simulink model "Ackermann_Env"  (R2025a)
settings: Solver=FixedStepAuto  StartTime=0.0  RelTol=1e-3
values from neighbouring files (symbols this model uses):
  dist0 = sqrt((pathXY_padded(end,1)-x0)^2 + (pathXY_padded(end,2)-y0)^2)    [testing_sebelum_v3.m]    (also in testing_v2.m)
  pathXY_padded = zeros(MAX_PATH_SIZE, 2)    [pad_path.m]    (also in pad_path_old.m = [pathXY; pad]; testing_sebelum_v3.m = pad_path(pathXY_raw, MAX_PATH_SIZE); testing_v2.m = pad_path(pathXY_raw, MAX_PATH_SIZE))
  slip_factor = 1.0    (= 1)    [testing_sebelum_v3.m]
undefined symbols (not defined in the file or in its folder): idx0
libraries: ros2lib x2, rllib x1
settings Model: Creator=raka-argha  LastModifiedBy=raka-argha
settings OptimizationCC: DefaultParameterBehavior=Inlined  EnhancedBackFolding=on  PassReuseOutputArgsAs=Individual arguments  ZeroExternalMemoryAtStartup=off  ZeroInternalMemoryAtStartup=off  MaxStackSize=64  OptimizeBlockOrder=speed  DifferentSizesBufferReuse=on  OptimizationCustomize=off  EfficientTunableParamExpr=on
settings DebuggingCC: ParameterTunabilityLossMsg=error
settings HardwareCC: ProdBitPerLong=64.0  ProdHWDeviceType=Intel->x86-64 (Linux 64)
settings SFSimCC: MATLABDynamicMemAlloc=off
settings RTWCC: SystemTargetFile=ert.tlc  HardwareBoard=Robot Operating System 2 (ROS 2)  TLCOptions="-aInlineSetEventsForThisBaseRateFcn=TLC_FALSE -aSuppressMultiTaskScheduler=TLC_FALSE  -aRateBasedStepFcn=0"  TemplateMakefile=ert_default_tmf  Toolchain=Colcon Tools  TargetLang=C++  Description=Embedded Coder
settings CodeAppCC: ForceParamTrailComments=on  IgnoreCustomStorageClasses=off  OperatorAnnotations=on  SimulinkDataObjDesc=on  SFDataObjDesc=on  InsertBlockDesc=on
settings ERTTargetCC: ExtModeTransport=2.0  RootIOFormat=Structure reference  CodeInterfacePackaging=C++ class

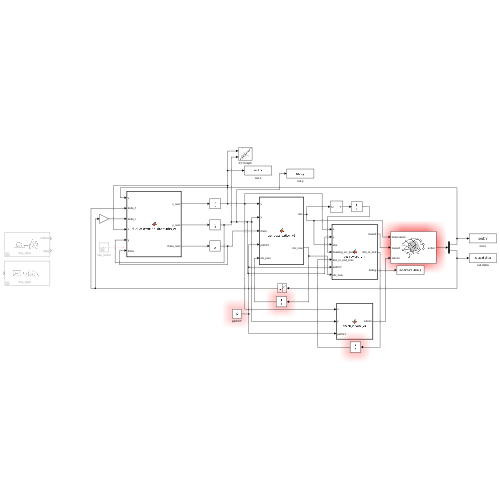
[thumbnail: Simulink's stored preview of the top-level diagram]
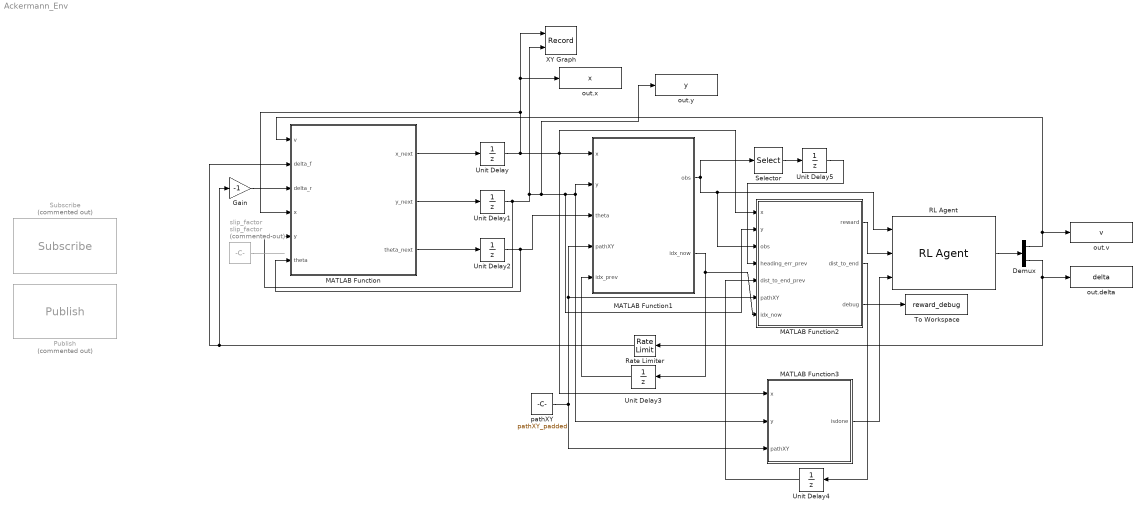
== system Ackermann_Env ==
  Demux : Demux  Outputs=2
  Gain : Gain  Gain=-1
  MATLAB Function : MATLAB Function  TreatAsAtomicUnit=on
  MATLAB Function1 : MATLAB Function  TreatAsAtomicUnit=on
  MATLAB Function2 : MATLAB Function  TreatAsAtomicUnit=on
  MATLAB Function3 : MATLAB Function  TreatAsAtomicUnit=on
  Publish : ros2lib/Publish  Commented=on  topicSource=Select from ROS network  topic=/my_topic  messageType=geometry_msgs/Point  QOSHistory=Keep last  QOSDepth=10  QOSReliability=Reliable  QOSDurability=Volatile  QOSDeadline=Inf  QOSLifespan=Inf  QOSLiveliness=Automatic  QOSLeaseDuration=Inf  QOSAvoidROSNamespaceConventions=off
  RL Agent : rllib/RL Agent  Agent=agentObj  ExternalActionAsInput=off  ProvideLastAction=off  ProvideCumRwd=off  TreatAsDirectFeedthrough=on  UseStrictObservationDataTypes=off
  Rate Limiter : RateLimiter  RisingSlewLimit=1.0  FallingSlewLimit=-1.0  SampleTimeMode=inherited
  Selector : Selector  IndexOptions=Index vector (dialog)  Indices=2  OutputSizes=1
  Subscribe : ros2lib/Subscribe  Commented=on  topicSource=Select from ROS network  topic=/my_topic  messageType=geometry_msgs/Point  sampleTime=-1  QOSHistory=Keep last  QOSDepth=10  QOSReliability=Reliable  QOSDurability=Volatile  QOSDeadline=Inf  QOSLifespan=Inf  QOSLiveliness=Automatic  QOSLeaseDuration=Inf  QOSAvoidROSNamespaceConventions=off
  To Workspace : ToWorkspace  VariableName=reward_debug  SaveFormat=Timeseries  SampleTime=-1
  Unit Delay{,1..2,5} (4 alike) : UnitDelay  SampleTime=-1  HasFrameUpgradeWarning=on
  Unit Delay3 : UnitDelay  InitialCondition=idx0  SampleTime=-1  HasFrameUpgradeWarning=on
  Unit Delay4 : UnitDelay  InitialCondition=dist0  SampleTime=-1  HasFrameUpgradeWarning=on
  XY Graph : Record  NumPorts=2.0  FileSettingsInternal="{\"entries\":[{\"content\":{\"excelSettings\":{\"content\":{},\"type\":\"Streamout.ExcelSettings\"},\"parquetSettings\":{\"content\":{},\"type\":\"Streamout.ParquetSettings\"}},\"type\":\"Streamout.FileSettingStorage\",\"uuid\":\"\"}],\"packageUris\":[\"http:\\/\\/schema.mathworks.com\\/mf0\\/streamout_blocks\\/R2020a\"],\"version\":\"1.0\"}"  FrameSettings=[0, 0]  Layout=[1 1]  SignalsInternal="{\"entries\":[{\"content\":{\"signals\":[{\"content\":{\"blockPath\":[],\"dimensions\":[1],\"domain\":\"\",\"lineColor\":\"#fe330a\",\"lineWidth\":2,\"port\":1,\"signalID\":1,\"signalName\":\"Unit Delay\"},\"type\":\"RecordBlkView.Signal\",\"uuid\":\"\"},{\"content\":{\"blockPath\":[],\"dimensions\":[1],\"domain\":\"\",\"lineColor\":\"#22b573\",\"lineWidth\":2,\"port\":2,\"signalID\":2,\"signalName\":\"Unit Delay1\"},\"type\":\"RecordBlkView.Signal\",\"uuid\":\"\"}]},\"type\":\"RecordBlkView.InputSignals\",\"uuid\":\"\"}],\"packageUris\":[\"http:\\/\\/schema.mathworks.com\\/mf0\\/streamout_blocks\\/R2020a\"],\"version\":\"1.0\"}"  VisualizationBindings="{\"xyplotplugin\":{\"info\":[{\"series\":[],\"subplotID\":1}]}}"  CompatibilityTag=XY
  out.delta : ToWorkspace  VariableName=delta  SaveFormat=Timeseries  SampleTime=-1
  out.v : ToWorkspace  VariableName=v  SaveFormat=Timeseries  SampleTime=-1
  out.x : ToWorkspace  VariableName=x  SaveFormat=Timeseries  SampleTime=-1
  out.y : ToWorkspace  VariableName=y  SaveFormat=Timeseries  SampleTime=-1
  pathXY : Constant  Value=pathXY_padded
  slip_factor : Constant  Commented=on  Value=slip_factor
  wires:
  MATLAB Function/1(x_next) -> Unit Delay/1
  MATLAB Function/2(y_next) -> Unit Delay1/1
  MATLAB Function/3(theta_next) -> Unit Delay2/1
  Unit Delay/1 -> out.x/1, XY Graph/1, MATLAB Function/4(x), MATLAB Function3/1(x), MATLAB Function2/1(x), MATLAB Function1/1(x)
  Unit Delay1/1 -> XY Graph/2, out.y/1, MATLAB Function2/2(y), MATLAB Function3/2(y), MATLAB Function1/2(y), MATLAB Function/5(y)
  Unit Delay2/1 -> MATLAB Function1/3(theta), MATLAB Function/6(theta)
  MATLAB Function1/1(obs) -> RL Agent/1, MATLAB Function2/3(obs), Selector/1
  MATLAB Function3/1(isdone) -> RL Agent/3
  MATLAB Function2/1(reward) -> RL Agent/2
  RL Agent/1 -> Demux/1
  Demux/1 -> out.v/1, MATLAB Function/1(v)
  Demux/2 -> Rate Limiter/1, out.delta/1
  Rate Limiter/1 -> Gain/1, MATLAB Function/2(delta_f)
  pathXY/1 -> MATLAB Function1/4(pathXY), MATLAB Function2/6(pathXY), MATLAB Function3/3(pathXY)
  Unit Delay4/1 -> MATLAB Function2/5(dist_to_end_prev)
  slip_factor/1 -> ?
  Selector/1 -> Unit Delay5/1
  MATLAB Function2/2(dist_to_end) -> Unit Delay4/1
  MATLAB Function2/3(debug) -> To Workspace/1
  Unit Delay5/1 -> MATLAB Function2/4(heading_err_prev)
  MATLAB Function1/2(idx_now) -> MATLAB Function2/7(idx_now), Unit Delay3/1
  Unit Delay3/1 -> MATLAB Function1/5(idx_prev)
  Gain/1 -> MATLAB Function/3(delta_r)

== matlab function Ackermann_Env/MATLAB Function1 ==
  data: x input; obs output; y input; theta input; pathXY input; idx_prev input; idx_now output
function [obs, idx_now] = get_observation_v6(x, y, theta, pathXY, idx_prev)
%#codegen
% GET_OBSERVATION_V6
%
% PERBEDAAN UTAMA DARI V5:
%   1. Index TIDAK BOLEH merayap melewati ujung path ASLI (N), bukan ujung
%      array padding (300). Ini yang dulu bikin dist_to_end jadi 0 permanen.
%   2. Observasi dinormalisasi supaya skalanya seragam (CTE ~1, waypoint ~5m
%      dibagi 5). SAC jauh lebih stabil dengan input yang sebanding.
%
% Ukuran port TIDAK BERUBAH: 5 input, 2 output, obs tetap 23x1.
% Jadi TIDAK PERLU mengubah wiring Simulink sama sekali.

    N_LOOKAHEAD = 10;
    STRIDE      = 5;
    WINDOW_BACK = 2;
    WINDOW_FWD  = 5;
    SKALA_WP    = 5.0;    % waypoint lookahead dibagi ini

    N = panjang_path_asli(pathXY);

    idx_prev = round(idx_prev);
    if idx_prev < 1, idx_prev = 1; end
    if idx_prev > N, idx_prev = N; end

    lo = max(1, idx_prev - WINDOW_BACK);
    hi = min(N, idx_prev + WINDOW_FWD);

    best_d = inf;
    best_i = idx_prev;
    for i = lo:hi
        d = (pathXY(i,1)-x)^2 + (pathXY(i,2)-y)^2;
        if d < best_d
            best_d = d;
            best_i = i;
        end
    end
    idx_now = best_i;
    dist_nearest = sqrt(best_d);

    % arah path di titik idx_now (pakai segmen mundur kalau sudah di ujung,
    % supaya tidak pernah atan2(0,0) di daerah padding)
    if idx_now < N
        seg_dx = pathXY(idx_now+1,1) - pathXY(idx_now,1);
        seg_dy = pathXY(idx_now+1,2) - pathXY(idx_now,2);
    elseif N > 1
        seg_dx = pathXY(N,1) - pathXY(N-1,1);
        seg_dy = pathXY(N,2) - pathXY(N-1,2);
    else
        seg_dx = 1; seg_dy = 0;
    end
    theta_path = atan2(seg_dy, seg_dx);

    heading_err = theta - theta_path;
    heading_err = atan2(sin(heading_err), cos(heading_err));

    to_robot_x = x - pathXY(idx_now,1);
    to_robot_y = y - pathXY(idx_now,2);
    CTE = -sin(theta_path)*to_robot_x + cos(theta_path)*to_robot_y;

    rel_wp = zeros(2*N_LOOKAHEAD, 1);
    ct = cos(-theta); st = sin(-theta);
    for k = 1:N_LOOKAHEAD
        idx_k = min(idx_now + k*STRIDE, N);       % dibatasi N, bukan M
        gx = pathXY(idx_k,1) - x;
        gy = pathXY(idx_k,2) - y;
        lx = ct*gx - st*gy;
        ly = st*gx + ct*gy;
        rel_wp(2*k-1) = lx / SKALA_WP;
        rel_wp(2*k)   = ly / SKALA_WP;
    end

    % CATATAN untuk get_reward_v11:
    %   obs(1) = CTE dalam METER (tidak dinormalisasi)
    %   obs(2) = heading_err dibagi pi  -> rentang [-1, 1]
    %   obs(3) = jarak ke titik path terdekat dalam METER
    obs = [CTE; heading_err/pi; dist_nearest; rel_wp];
end

% -------------------------------------------------------------------------
function N = panjang_path_asli(pathXY)
%#codegen
% Mengembalikan index titik terakhir path ASLI. Padding dibuat dengan cara
% mengulang titik terakhir (lihat pad_path.m), jadi titik-titik padding
% jaraknya nol dari titik sebelumnya.
    M = size(pathXY,1);
    N = 1;
    for i = M:-1:2
        dx = pathXY(i,1) - pathXY(i-1,1);
        dy = pathXY(i,2) - pathXY(i-1,2);
        if (dx*dx + dy*dy) > 1e-12
            N = i;
            return;
        end
    end
end

== matlab function Ackermann_Env/MATLAB Function ==
  data: v input; x_next output; delta_f input; delta_r input; x input; y input; theta input; y_next output; theta_next output
function [x_next, y_next, theta_next] = dual_ackermann_kinematics_v4(v, delta_f, delta_r, x, y, theta)
%#codegen
% DUAL_ACKERMANN_KINEMATICS_V4
% Sama seperti v3, TAPI slip_factor DIHAPUS TOTAL. Simulasi sekarang
% idealized murni (traksi sempurna). Slip akan dimodelkan nanti di
% simulasi 3D, bukan di sini.
%
% PORT BERUBAH: 6 input (dulu 7), 3 output.
% Di Simulink: HAPUS port input 'slip_factor' pada blok ini, dan HAPUS
% blok Constant 'slip_factor' di level Ackermann_Env.
%
% Kinematika bodi 4 roda, kemudi depan DAN belakang, diturunkan dari ICR:
%   delta_r = -delta_f  -> dual Ackermann simetris (R_min terkecil)
%   delta_r = 0         -> Ackermann biasa (setir depan saja)
%   delta_r = +delta_f  -> CRAB (translasi menyamping, tanpa berputar)
%
%   b = L / (tan(df) - tan(dr))      <- ICR koordinat y
%   a = L/2 - b*tan(df)              <- ICR koordinat x
%   kecepatan titik tengah = omega*(b, -a), besarnya = v

    p  = robot_params();
    L  = p.L;
    Ts = 0.1;
    EPS = 1e-6;

    tf = tan(delta_f);
    tr = tan(delta_r);
    denom = tf - tr;

    if abs(denom) < EPS
        % tidak ada rotasi: lurus (df=dr=0) atau crab (df=dr=c)
        omega = 0;
        vx_b  = v * cos(delta_f);
        vy_b  = v * sin(delta_f);
    else
        b = L / denom;
        a = L/2 - b*tf;
        r_c = sqrt(a*a + b*b);

        omega = sign(b) * v / r_c;
        vx_b  = omega * b;
        vy_b  = omega * (-a);   % NOL saat simetris; tidak nol = menyamping
    end

    ct = cos(theta); st = sin(theta);
    x_next     = x + (vx_b*ct - vy_b*st) * Ts;
    y_next     = y + (vx_b*st + vy_b*ct) * Ts;
    theta_next = theta + omega * Ts;
    theta_next = atan2(sin(theta_next), cos(theta_next));
end

== matlab function Ackermann_Env/MATLAB Function2 ==
  data: x input; y input; obs input; reward output; heading_err_prev input; dist_to_end_prev input; pathXY input; dist_to_end output; debug output; idx_now input
function [reward, dist_to_end, debug] = get_reward_v11(x, y, obs, heading_err_prev, dist_to_end_prev, pathXY, idx_now)
%#codegen
% GET_REWARD_V11
%
% PERUBAHAN PALING PENTING vs v9/v10:
%   r_goal TIDAK LAGI memakai dist_to_end (panjang busur dari index).
%   r_goal memakai JARAK EUCLIDEAN ASLI dari (x,y) ke titik akhir path asli
%   -- rumus yang PERSIS SAMA dengan check_isdone_v4. Jadi secara matematis
%   mustahil r_goal menyala tanpa episode ikut berhenti.
%
%   Konsekuensinya: batas atas reward satu episode sekarang terhitung.
%   400 step x 10 (clamp) + 300 (goal) = 4300. Kalau kamu masih melihat
%   angka 10.000+, berarti ada masalah LAIN dan itu langsung ketahuan.
%
% Ukuran port TIDAK BERUBAH: 7 input, 3 output. debug melebar dari 6 ke 8
% elemen (Simulink menyesuaikan sendiri, tidak perlu rewiring).

    % --- baca observasi (skala harus cocok dengan get_observation_v6) ---
    CTE          = obs(1);          % meter
    heading_err  = obs(2);          % sudah dibagi pi, rentang [-1,1]
    dist_nearest = obs(3);          % meter

    N = panjang_path_asli(pathXY);

    idxn = round(idx_now);
    if idxn < 1, idxn = 1; end
    if idxn > N, idxn = N; end

    % --- panjang busur sisa (HANYA untuk progress shaping, BUKAN untuk goal) ---
    dist_to_end = 0;
    for i = idxn : N-1
        dx = pathXY(i+1,1) - pathXY(i,1);
        dy = pathXY(i+1,2) - pathXY(i,2);
        dist_to_end = dist_to_end + sqrt(dx*dx + dy*dy);
    end

    % --- progress: robot maks 0.1 m/step, jadi clamp 0.5 sudah sangat longgar ---
    raw_progress = dist_to_end_prev - dist_to_end;
    raw_progress = max(-0.5, min(0.5, raw_progress));
    r_progress = 30.0 * raw_progress;

    % --- yaw improvement (dua-duanya dalam satuan ternormalisasi) ---
    yaw_improve = abs(heading_err_prev) - abs(heading_err);
    yaw_improve = max(-0.2, min(0.2, yaw_improve));
    r_yaw = 15.0 * yaw_improve;

    % --- jaga tetap dekat path ---
    r_cte = -6.0 * abs(CTE);

    step_penalty = -0.05;

    shaped = r_progress + r_yaw + r_cte + step_penalty;
    shaped = max(-25, min(25, shaped));

    % --- GOAL: pakai jarak asli, identik dengan check_isdone_v4 ---
    p  = robot_params();
    Ng = max(1, N - p.n_ghost);        % tujuan ASLI, bukan ujung hantu
    dx_g = x - pathXY(Ng,1);
    dy_g = y - pathXY(Ng,2);
    d_goal = sqrt(dx_g*dx_g + dy_g*dy_g);

    r_goal = 0;
    if d_goal < 0.3
        r_goal = 300;
    end

    % --- KELUAR JALUR: identik dengan check_isdone_v4 ---
    r_off = 0;
    if dist_nearest > 0.5
        r_off = -100;
    end

    reward = shaped + r_goal + r_off;

    debug = [r_progress; r_yaw; r_cte; r_goal; r_off; reward; double(idxn); d_goal];
end

% -------------------------------------------------------------------------
function N = panjang_path_asli(pathXY)
%#codegen
    M = size(pathXY,1);
    N = 1;
    for i = M:-1:2
        dx = pathXY(i,1) - pathXY(i-1,1);
        dy = pathXY(i,2) - pathXY(i-1,2);
        if (dx*dx + dy*dy) > 1e-12
            N = i;
            return;
        end
    end
end

== matlab function Ackermann_Env/MATLAB Function3 ==
  data: x input; y input; pathXY input; isdone output
function isdone = check_isdone_v4(x, y, pathXY)
%#codegen
% CHECK_ISDONE_V4
%
% Tiga syarat berhenti:
%   1. SAMPAI   : jarak asli ke titik akhir < 0.3 m   (cocok dengan r_goal)
%   2. NYASAR   : jarak ke titik path terdekat > 1.5 m (cocok dengan r_off)
%   3. KABUR    : posisi di luar kotak +-50 m (pengaman numerik)
%
% Syarat ke-2 adalah yang membunuh exploit "robot muter-muter": dulu robot
% bisa berputar 400 step dan mengisi replay buffer dengan sampah. Sekarang
% episodenya dipotong dalam beberapa step.
%
% Sengaja TIDAK menambah port input: jarak ke path dihitung sendiri di sini
% dengan scan penuh (bukan windowed), jadi tidak bisa tertipu index yang
% merayap. Ukuran port tetap 3 input / 1 output -> tanpa rewiring.

    N = panjang_path_asli(pathXY);

    % 1. sampai tujuan
    p  = robot_params();
    Ng = max(1, N - p.n_ghost);        % tujuan ASLI, bukan ujung hantu
    dx_g = x - pathXY(Ng,1);
    dy_g = y - pathXY(Ng,2);
    d_goal = sqrt(dx_g*dx_g + dy_g*dy_g);

    % 2. jarak ke path terdekat (scan seluruh path asli)
    best = inf;
    for i = 1:N
        dx = pathXY(i,1) - x;
        dy = pathXY(i,2) - y;
        d = dx*dx + dy*dy;
        if d < best
            best = d;
        end
    end
    d_path = sqrt(best);

    if (d_goal < 0.3) || (d_path > 0.5) || (abs(x) > 50) || (abs(y) > 50)
        isdone = 1;
    else
        isdone = 0;
    end
end

% -------------------------------------------------------------------------
function N = panjang_path_asli(pathXY)
%#codegen
    M = size(pathXY,1);
    N = 1;
    for i = M:-1:2
        dx = pathXY(i,1) - pathXY(i-1,1);
        dy = pathXY(i,2) - pathXY(i-1,2);
        if (dx*dx + dy*dy) > 1e-12
            N = i;
            return;
        end
    end
end
